simulink model "cgex"  (R2018b)
settings: Solver=FixedStepDiscrete  StartTime=0.0  StopTime=10.0  FixedStep=0.01  RelTol=1e-3
values from neighbouring files (symbols this model uses):
  k = 2.0    [ggexdd.sldd]
settings Model: DataDictionary=ggexdd.sldd  Creator=19810  LastModifiedBy=19810
settings OptimizationCC: DefaultParameterBehavior=Inlined  EnhancedBackFolding=on  PassReuseOutputArgsAs=Individual arguments  OptimizeBlockOrder=speed  DifferentSizesBufferReuse=on  OptimizationCustomize=off
settings DebuggingCC: ParameterTunabilityLossMsg=error
settings SFSimCC: MATLABDynamicMemAlloc=off
settings RTWCC: SystemTargetFile=ert.tlc  TemplateMakefile=ert_default_tmf  GenerateReport=on  IncludeHyperlinkInReport=on  LaunchReport=on  GenerateTraceInfo=on  GenerateTraceReport=on  GenerateTraceReportSl=on  GenerateTraceReportSf=on  GenerateTraceReportEml=on
settings CodeAppCC: ForceParamTrailComments=on  IgnoreCustomStorageClasses=off  OperatorAnnotations=on  SimulinkDataObjDesc=on  SFDataObjDesc=on  InsertBlockDesc=on
settings ERTTargetCC: TargetLangStandard=C99 (ISO)  GenerateSampleERTMain=on  InlinedParameterPlacement=NonHierarchical  ERTCustomFileTemplate=example_file_process.tlc

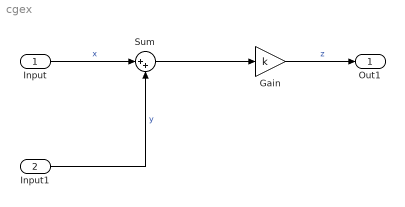
== system cgex ==
  Input : Inport
  Input1 : Inport  Port=2
  Gain : Gain  Gain=k
  Sum : Sum  Inputs=|++
  Out1 : Outport
  wires:
  Input/1 -> Sum/1  "x"
  Input1/1 -> Sum/2  "y"
  Sum/1 -> Gain/1
  Gain/1 -> Out1/1  "z"
